simulink model "part1_pendulum_regulation_R2021a"  (R2021a)
settings: Solver=ode45  StartTime=0.0  StopTime=2  MaxStep=0.005  RelTol=1e-8  AbsTol=1e-10
model workspace (MAT data in the model file):
  Kd = 12
  Kp = 36
  g = 9.81
  k = 0.05
  l = 0.5
  m = 0.2
  omega0 = 0
  theta0 = 0.1
settings Model: Creator=matiasgarcia  LastModifiedBy=matiasgarcia
settings DataIOCC: SaveOutput=off  SignalLogging=off  SaveTime=off
settings DebuggingCC: UnconnectedInputMsg=none  UnconnectedOutputMsg=none  UnconnectedLineMsg=none
settings ModelReferenceCC: EnableRefExpFcnMdlSchedulingChecks=off
settings RTWCC: Description=Generic Real-Time Target  GPUComputeCapability=5.0  DLArmComputeVersion=20.02.1

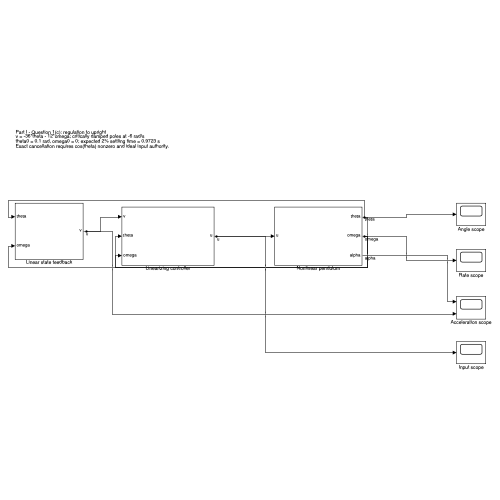
[thumbnail: Simulink's stored preview of the top-level diagram]
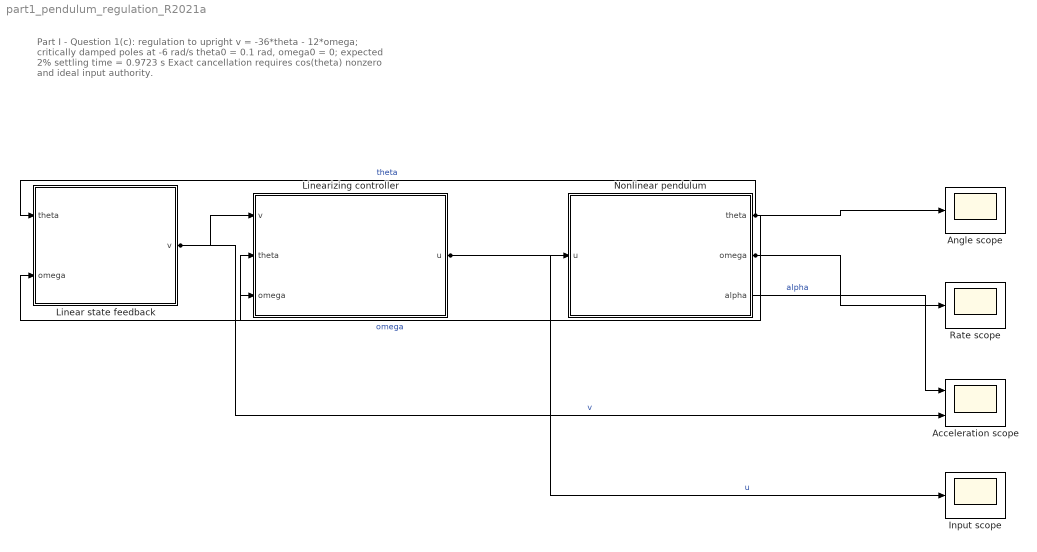
== system part1_pendulum_regulation_R2021a ==
  note: Part I - Question 1(c): regulation to upright
      | v = -36*theta - 12*omega; critically damped poles at -6 rad/s
      | theta0 = 0.1 rad, omega0 = 0; expected 2% settling time = 0.9723 s
      | Exact cancellation requires cos(theta) nonzero and ideal input authority.
  Acceleration scope : Scope  NumInputPorts=2
  Angle scope : Scope
  Input scope : Scope
  Linear state feedback : Subsystem
  Linearizing controller : Subsystem
  Nonlinear pendulum : Subsystem
  Rate scope : Scope
  wires:
  Nonlinear pendulum/1(theta) -> Linearizing controller/2(theta), Angle scope/1, Linear state feedback/1(theta)  "theta"
  Nonlinear pendulum/2(omega) -> Linearizing controller/3(omega), Rate scope/1, Linear state feedback/2(omega)  "omega"
  Linearizing controller/1(u) -> Nonlinear pendulum/1(u), Input scope/1  "u"
  Nonlinear pendulum/3(alpha) -> Acceleration scope/1  "alpha"
  Linear state feedback/1(v) -> Linearizing controller/1(v), Acceleration scope/2  "v"

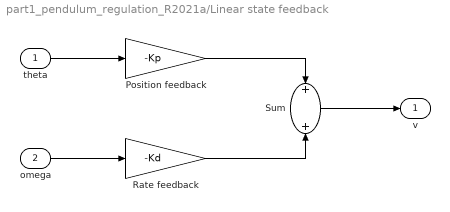
== system part1_pendulum_regulation_R2021a/Linear state feedback ==
  theta : Inport
  omega : Inport  Port=2
  Position feedback : Gain  Gain=-Kp
  Rate feedback : Gain  Gain=-Kd
  Sum : Sum
  v : Outport
  wires:
  theta/1 -> Position feedback/1
  omega/1 -> Rate feedback/1
  Position feedback/1 -> Sum/1
  Rate feedback/1 -> Sum/2
  Sum/1 -> v/1

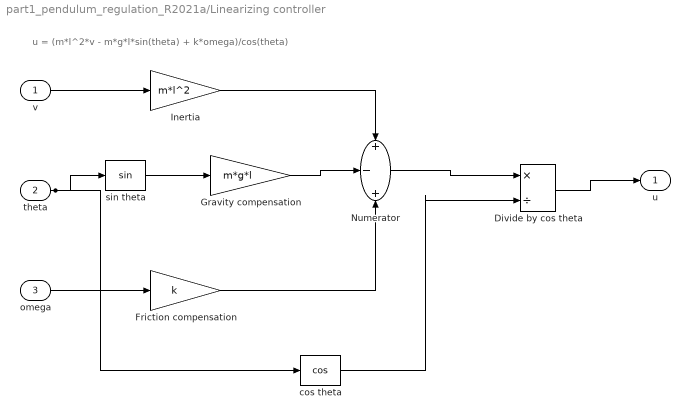
== system part1_pendulum_regulation_R2021a/Linearizing controller ==
  note: u = (m*l^2*v - m*g*l*sin(theta) + k*omega)/cos(theta)
  v : Inport
  theta : Inport  Port=2
  omega : Inport  Port=3
  Divide by cos theta : Product  Inputs=*/
  Friction compensation : Gain  Gain=k
  Gravity compensation : Gain  Gain=m*g*l
  Inertia : Gain  Gain=m*l^2
  Numerator : Sum  Inputs=+-+
  cos theta : Trigonometry  Operator=cos
  sin theta : Trigonometry
  u : Outport
  wires:
  v/1 -> Inertia/1
  theta/1 -> sin theta/1, cos theta/1
  sin theta/1 -> Gravity compensation/1
  omega/1 -> Friction compensation/1
  Inertia/1 -> Numerator/1
  Gravity compensation/1 -> Numerator/2
  Friction compensation/1 -> Numerator/3
  Numerator/1 -> Divide by cos theta/1
  cos theta/1 -> Divide by cos theta/2
  Divide by cos theta/1 -> u/1

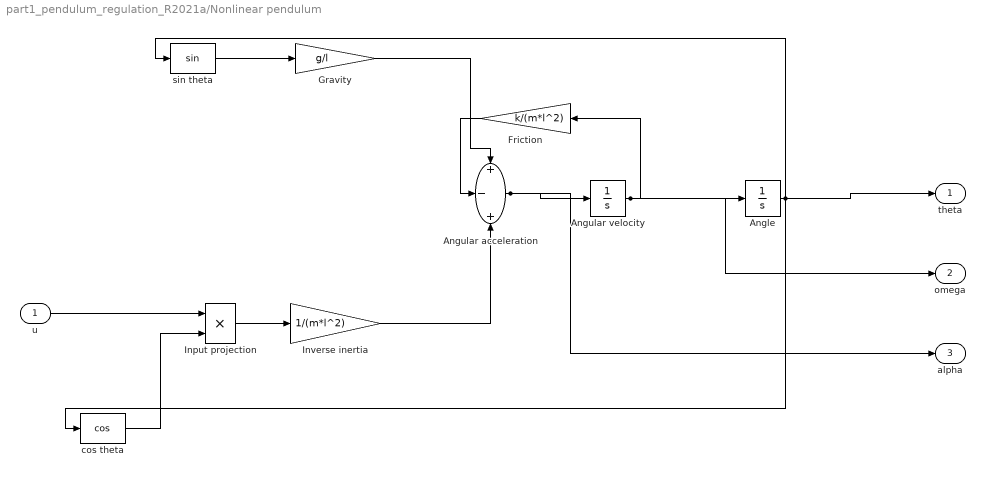
== system part1_pendulum_regulation_R2021a/Nonlinear pendulum ==
  u : Inport
  Angle : Integrator  InitialCondition=theta0
  Angular acceleration : Sum  Inputs=+-+
  Angular velocity : Integrator  InitialCondition=omega0
  Friction : Gain  Gain=k/(m*l^2)
  Gravity : Gain  Gain=g/l
  Input projection : Product
  Inverse inertia : Gain  Gain=1/(m*l^2)
  cos theta : Trigonometry  Operator=cos
  sin theta : Trigonometry
  theta : Outport
  omega : Outport  Port=2
  alpha : Outport  Port=3
  wires:
  u/1 -> Input projection/1
  cos theta/1 -> Input projection/2
  Input projection/1 -> Inverse inertia/1
  Inverse inertia/1 -> Angular acceleration/3
  sin theta/1 -> Gravity/1
  Gravity/1 -> Angular acceleration/1
  Angular velocity/1 -> Friction/1, Angle/1, omega/1
  Friction/1 -> Angular acceleration/2
  Angular acceleration/1 -> Angular velocity/1, alpha/1
  Angle/1 -> sin theta/1, cos theta/1, theta/1
